simulink model "QuadcopterSimModel_Loiter_FTC_dseg"  (R2026a)
settings: Solver=ode2  StartTime=-5  StopTime=25  FixedStep=1/800  RelTol=1e-4  EnableMultiTasking=on
undefined symbols (not defined in the file): alt_ground, atmosphere, dseg_stop_en, envir, failure_time_mot_1, failure_time_mot_2, failure_time_mot_3, failure_time_mot_4, ffpar, g, pos_ref, westpar, wind
libraries: unit_conversions_lib x3, flightgear_visualization_lib x2, copterFtc_lib x2, atmosphere_lib x1, sensors_lib x1, quadcopter_lib x1, axes_transformation_lib x1
settings Model: Creator=Yannic  LastModifiedBy=wngh2
settings SolverCC: ZeroCrossControl=DisableAll
settings OptimizationCC: EfficientMapNaN2IntZero=off
settings DebuggingCC: ReadBeforeWriteMsg=DisableAll  WriteAfterWriteMsg=DisableAll  WriteAfterReadMsg=DisableAll  MultiTaskDSMMsg=none  MultiTaskRateTransMsg=warning
settings HardwareCC: TargetBitPerPointer=64.0  TargetBitPerSizeT=64.0  TargetBitPerPtrDiffT=64.0  TargetLongLongMode=on  TargetIntDivRoundTo=Zero  TargetEndianess=LittleEndian  TargetWordSize=64.0  TargetHWDeviceType=MATLAB Host  ProdEqTarget=off
settings SFSimCC: SFSimEcho=off
settings CodeAppCC: MaxIdLength=128.0
settings GRTTargetCC: CombineOutputUpdateFcns=off  GRTInterface=on

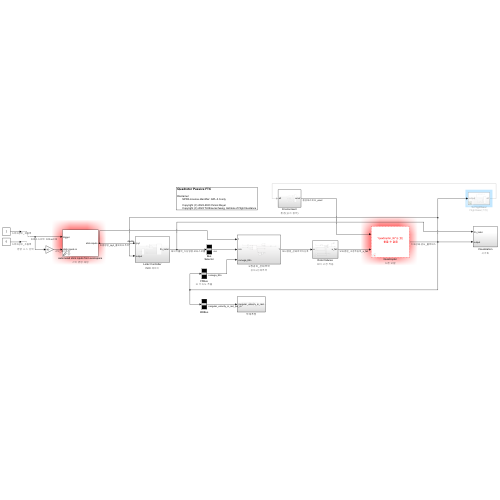
[thumbnail: Simulink's stored preview of the top-level diagram]
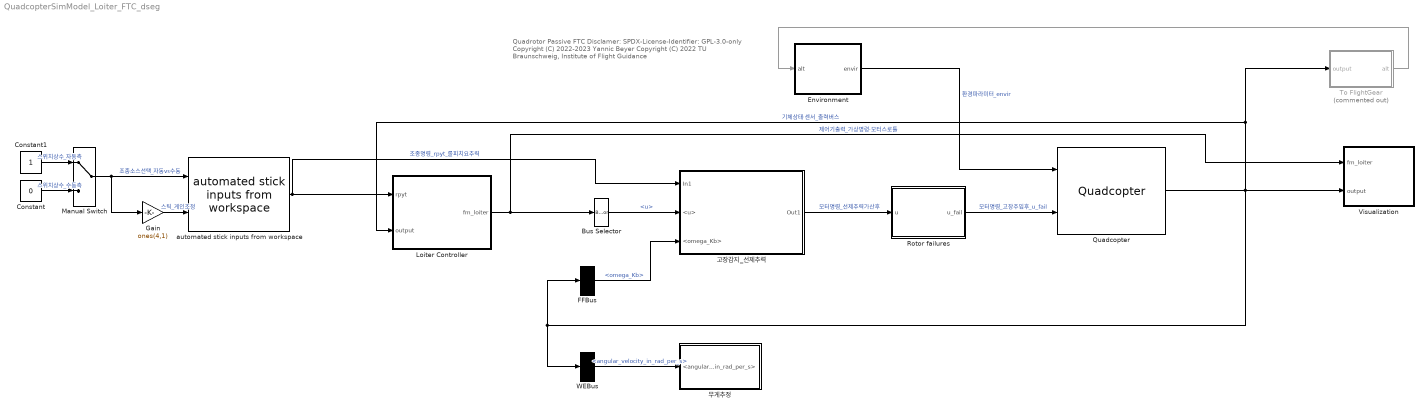
== system QuadcopterSimModel_Loiter_FTC_dseg ==
  note: Quadrotor Passive FTC
      |
      | Disclamer:
      | SPDX-License-Identifier: GPL-3.0-only
      |
      | Copyright (C) 2022-2023 Yannic Beyer
      | Copyright (C) 2022 TU Braunschweig, Institute of Flight Guidance
  Bus Selector : BusSelector  OutputSignals=inner_loop_indi.u
  Constant : Constant  Value=0
  Constant1 : Constant
  Environment : Subsystem  Description=고도 → 공기밀도·중력 등 환경 버스 계산
      settings: AttributesFormatString=환경(공기·중력)
  FFBus : BusSelector  Description=드론 상태 버스에서 요 각속도(omega_Kb) 추출 → 감지기로  OutputSignals=rigidBodyBus.omega_Kb
      settings: AttributesFormatString=요 각속도 추출
  Gain : Gain  Gain=ones(4,1)
  Loiter Controller : Subsystem  Description=INDI 로이터 제어기. 명령 + 피드백 → 모터 명령
      settings: AttributesFormatString=INDI 제어기
  Manual Switch : ManualSwitch  Description=명령 소스 선택 (sw=1: 자동 스틱 사용)
      settings: AttributesFormatString=명령 소스 선택
  Quadcopter : quadcopter_lib/Quadcopter  Description=드론 모델(동역학). 모터명령 → 힘·모멘트 → 상태(위치·자세·각속도)  copter_=copter  IC_=IC  grnd_=grnd
      settings: AttributesFormatString=드론 모델  SourceProductName=Quadcopter
  Rotor failures : Subsystem  Description=failure_time_mot_* 에 지정된 모터를 그 시각에 정지(스로틀 0)
      settings: AttributesFormatString=모터 고장 적용
  To FlightGear : Subsystem  Description=FlightGear 연동 (주석처리 — MATLAB Coder 필요)  Commented=on
      settings: AttributesFormatString=FlightGear(꺼짐)
  Visualization : Subsystem  Description=상태 시각화 출력
      settings: AttributesFormatString=시각화
  WEBus : BusSelector  OutputSignals=motorBus.angular_velocity_in_rad_per_s
  automated stick inputs from workspace : copterFtc_lib/automated stick inputs from workspace  Description=스틱 명령(simin) 재생 → rpyt 4채널(롤·피치·요·스로틀)  simin=simin
      settings: AttributesFormatString=스틱 명령 재생
  고장감지_선제추력 : Subsystem  Description=요 추종오차로 고장 감지 → 잔여 모터에 선제추력 주입 (감지·판단·주입 한 묶음)
      settings: AttributesFormatString=감지+선제추력
  무게추정 : Subsystem
  wires:
  Environment/1(envir) -> Quadcopter/1  "환경파라미터_envir"
  Quadcopter/1 -> To FlightGear/1(output), Loiter Controller/2(output), Visualization/2(output), FFBus/1, WEBus/1  "기체상태·센서_출력버스"
  To FlightGear/1(alt) -> Environment/1(alt)
  Rotor failures/1(u_fail) -> Quadcopter/2  "모터명령_고장주입후_u_fail"
  Loiter Controller/1(fm_loiter) -> Visualization/1(fm_loiter), Bus Selector/1  "제어기출력_가상명령·모터스로틀"
  automated stick inputs from workspace/1 -> 고장감지_선제추력/1(In1), Loiter Controller/1(rpyt)  "조종명령_rpyt_롤피치요추력"
  Constant1/1 -> Manual Switch/1  "스위치상수_자동측"
  Manual Switch/1 -> Gain/1, automated stick inputs from workspace/1  "조종소스선택_자동vs수동"
  Constant/1 -> Manual Switch/2  "스위치상수_수동측"
  Gain/1 -> automated stick inputs from workspace/2  "스틱_게인조정"
  Bus Selector/1 -> 고장감지_선제추력/2(<u>)  "<u>"
  FFBus/1 -> 고장감지_선제추력/3(<omega_Kb>)  "<omega_Kb>"
  고장감지_선제추력/1(Out1) -> Rotor failures/1(u)  "모터명령_선제추력가산후"
  WEBus/1 -> 무게추정/1(<angular_velocity_in_rad_per_s>)  "<angular_velocity_in_rad_per_s>"

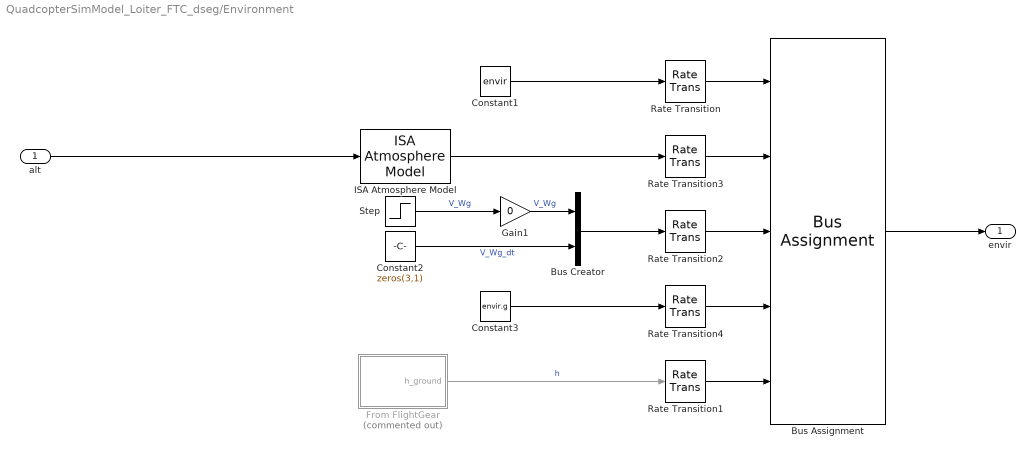
== system QuadcopterSimModel_Loiter_FTC_dseg/Environment ==
  alt : Inport
  Bus Assignment : BusAssignment  AssignedSignals=atmosphere,wind,g,alt_ground
  Bus Creator : BusCreator  Inputs=2
  Constant1 : Constant  Value=envir  OutDataTypeStr=Bus: envirBus
  Constant2 : Constant  Value=zeros(3,1)
  Constant3 : Constant  Value=envir.g
  From FlightGear : Subsystem  Commented=on
  Gain1 : Gain  Gain=0
  ISA Atmosphere Model : atmosphere_lib/ISA Atmosphere Model
      settings: SourceProductName=Atmosphere
  Rate Transition{,1..4} (5 alike) : RateTransition
  Step : Step  Time=3  FinalValue=[0;10;0]  SampleTime=0
  envir : Outport  VectorParamsAs1DForOutWhenUnconnected=off
  wires:
  From FlightGear/1(h_ground) -> Rate Transition1/1  "h"
  Rate Transition2/1 -> Bus Assignment/3
  Rate Transition3/1 -> Bus Assignment/2
  Bus Assignment/1 -> envir/1
  Rate Transition/1 -> Bus Assignment/1
  ISA Atmosphere Model/1 -> Rate Transition3/1
  Rate Transition1/1 -> Bus Assignment/5
  Constant1/1 -> Rate Transition/1
  alt/1 -> ISA Atmosphere Model/1
  Bus Creator/1 -> Rate Transition2/1
  Constant2/1 -> Bus Creator/2  "V_Wg_dt"
  Rate Transition4/1 -> Bus Assignment/4
  Constant3/1 -> Rate Transition4/1
  Gain1/1 -> Bus Creator/1  "V_Wg"
  Step/1 -> Gain1/1  "V_Wg"

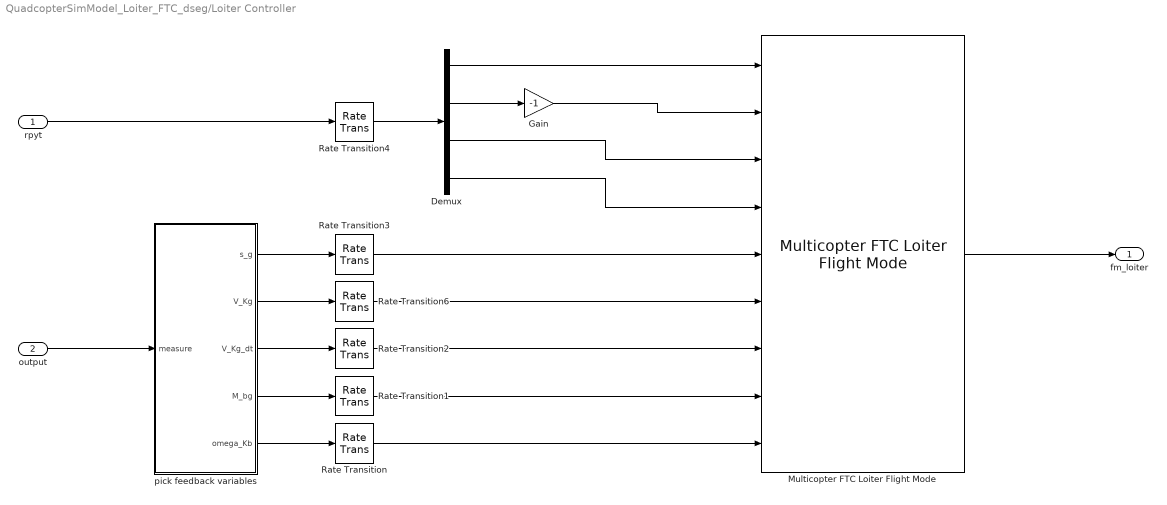
== system QuadcopterSimModel_Loiter_FTC_dseg/Loiter Controller ==
  rpyt : Inport  OutDataTypeStr=double
  output : Inport  Port=2
  Demux : Demux
  Gain : Gain  Gain=-1
  Multicopter FTC Loiter Flight Mode : copterFtc_lib/Multicopter FTC Loiter Flight Mode  fm=fm_loiter
  Rate Transition{,1..4,6} (6 alike) : RateTransition
  pick feedback variables : Subsystem
  fm_loiter : Outport  VectorParamsAs1DForOutWhenUnconnected=off
  wires:
  output/1 -> pick feedback variables/1(measure)
  rpyt/1 -> Rate Transition4/1
  Multicopter FTC Loiter Flight Mode/1 -> fm_loiter/1
  Demux/4 -> Multicopter FTC Loiter Flight Mode/4
  Demux/3 -> Multicopter FTC Loiter Flight Mode/3
  Demux/2 -> Gain/1
  Demux/1 -> Multicopter FTC Loiter Flight Mode/1
  Gain/1 -> Multicopter FTC Loiter Flight Mode/2
  Rate Transition4/1 -> Demux/1
  pick feedback variables/1(s_g) -> Rate Transition3/1
  pick feedback variables/5(omega_Kb) -> Rate Transition/1
  pick feedback variables/4(M_bg) -> Rate Transition1/1
  pick feedback variables/3(V_Kg_dt) -> Rate Transition2/1
  pick feedback variables/2(V_Kg) -> Rate Transition6/1
  Rate Transition/1 -> Multicopter FTC Loiter Flight Mode/9
  Rate Transition3/1 -> Multicopter FTC Loiter Flight Mode/5
  Rate Transition6/1 -> Multicopter FTC Loiter Flight Mode/6
  Rate Transition2/1 -> Multicopter FTC Loiter Flight Mode/7
  Rate Transition1/1 -> Multicopter FTC Loiter Flight Mode/8

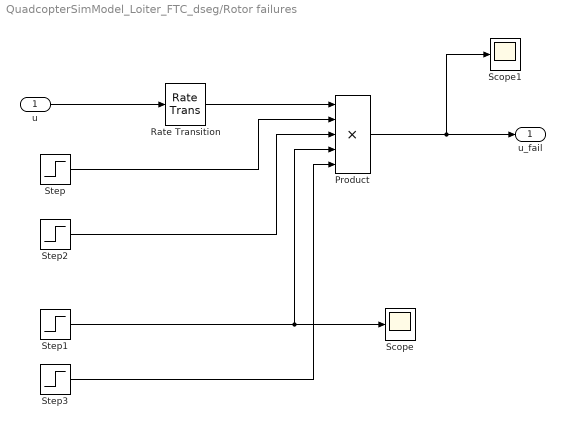
== system QuadcopterSimModel_Loiter_FTC_dseg/Rotor failures ==
  u : Inport
  Product : Product  Inputs=5
  Rate Transition : RateTransition
  Scope : Scope
      settings: ActiveDisplayYMinimum=-0.125  ActiveDisplayYMaximum=1.125  DataLoggingVariableName=ScopeData2
  Scope1 : Scope
      settings: ActiveDisplayYMinimum=-0.07201  ActiveDisplayYMaximum=0.64813
  Step : Step  Time=failure_time_mot_1  InitialValue=[1;1;1;1]  FinalValue=[0;1;1;1]  SampleTime=0
  Step1 : Step  Time=failure_time_mot_3  InitialValue=[1;1;1;1]  FinalValue=[1;1;0;1]  SampleTime=0
  Step2 : Step  Time=failure_time_mot_2  InitialValue=[1;1;1;1]  FinalValue=[1;0;1;1]  SampleTime=0
  Step3 : Step  Time=failure_time_mot_4  InitialValue=[1;1;1;1]  FinalValue=[1;1;1;0]  SampleTime=0
  u_fail : Outport  VectorParamsAs1DForOutWhenUnconnected=off
  wires:
  Product/1 -> Scope1/1, u_fail/1
  u/1 -> Rate Transition/1
  Rate Transition/1 -> Product/1
  Step1/1 -> Scope/1, Product/4
  Step2/1 -> Product/3
  Step/1 -> Product/2
  Step3/1 -> Product/5

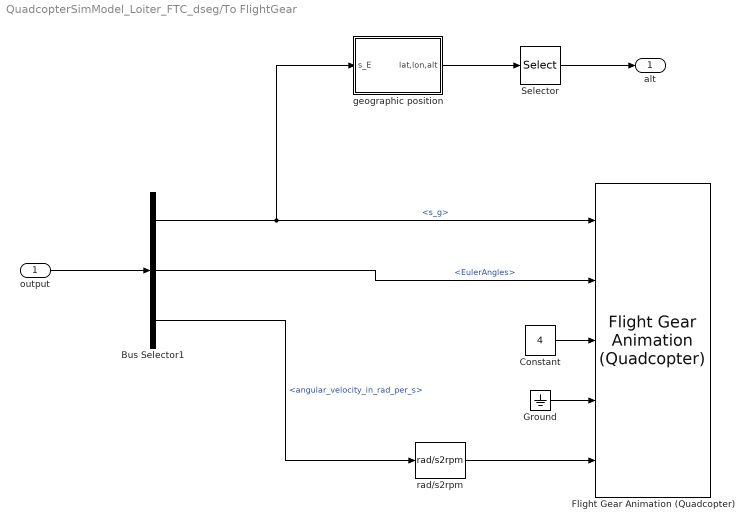
== system QuadcopterSimModel_Loiter_FTC_dseg/To FlightGear ==
  output : Inport
  Bus Selector1 : BusSelector  OutputSignals=rigidBodyBus.s_g,rigidBodyBus.EulerAngles,motorBus.angular_velocity_in_rad_per_s
  Constant : Constant  Value=4
  Flight Gear Animation (Quadcopter) : flightgear_visualization_lib/Flight Gear Animation (Quadcopter)  inital_lat=pos_ref.lat  inital_long=pos_ref.lon  inital_height=pos_ref.alt  remoteURL=fg.remoteURL  remotePort=fg.remotePort
      settings: SourceProductName=LADAC
  Ground : Ground
  Selector : Selector  InputPortWidth=3  IndexOptions=Index vector (dialog)  Indices=3  OutputSizes=1
  geographic position : Subsystem
  rad/s2rpm : unit_conversions_lib/rad//s2rpm
      settings: SourceProductName=LADAC
  alt : Outport  VectorParamsAs1DForOutWhenUnconnected=off
  wires:
  Bus Selector1/1 -> geographic position/1(s_E), Flight Gear Animation (Quadcopter)/1  "<s_g>"
  output/1 -> Bus Selector1/1
  geographic position/1(lat,lon,alt) -> Selector/1
  Bus Selector1/2 -> Flight Gear Animation (Quadcopter)/2  "<EulerAngles>"
  Bus Selector1/3 -> rad/s2rpm/1  "<angular_velocity_in_rad_per_s>"
  Selector/1 -> alt/1
  Constant/1 -> Flight Gear Animation (Quadcopter)/3
  Ground/1 -> Flight Gear Animation (Quadcopter)/4
  rad/s2rpm/1 -> Flight Gear Animation (Quadcopter)/5

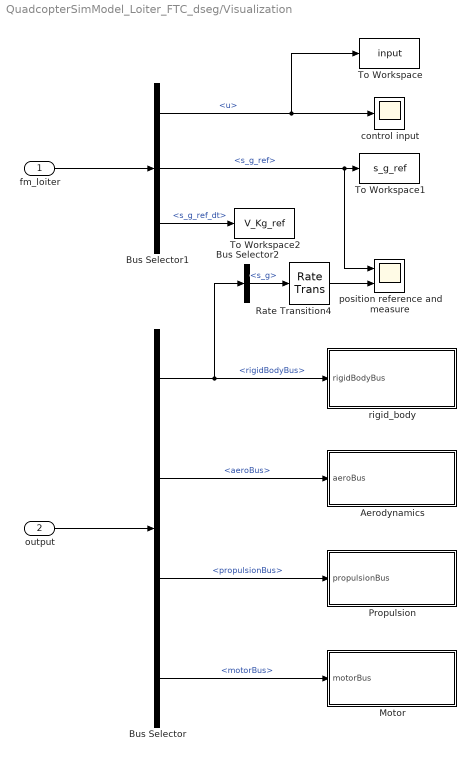
== system QuadcopterSimModel_Loiter_FTC_dseg/Visualization ==
  fm_loiter : Inport
  output : Inport  Port=2
  Aerodynamics : Subsystem
  Bus Selector : BusSelector  OutputSignals=rigidBodyBus,aeroBus,propulsionBus,motorBus
  Bus Selector1 : BusSelector  OutputSignals=inner_loop_indi.u,pos_cntrl.reference.s_g_ref,pos_cntrl.reference.s_g_ref_dt
  Bus Selector2 : BusSelector  OutputSignals=s_g
  Motor : Subsystem
  Propulsion : Subsystem
  Rate Transition4 : RateTransition
  To Workspace : ToWorkspace  VariableName=input  SaveFormat=Timeseries  SampleTime=-1
  To Workspace1 : ToWorkspace  VariableName=s_g_ref  SaveFormat=Timeseries  SampleTime=-1
  To Workspace2 : ToWorkspace  VariableName=V_Kg_ref  SaveFormat=Timeseries  SampleTime=-1
  control input : Scope
      settings: ActiveDisplayYMinimum=-0.0125  ActiveDisplayYMaximum=1.1125  DataLoggingVariableName=input
  position reference and measure : Scope  NumInputPorts=2
      settings: ActiveDisplayYMinimum=-0.60348  ActiveDisplayYMaximum=3.15627  DataLoggingVariableName=pos
  rigid_body : Subsystem
  wires:
  output/1 -> Bus Selector/1
  Bus Selector/1 -> Bus Selector2/1, rigid_body/1(rigidBodyBus)  "<rigidBodyBus>"
  Bus Selector/2 -> Aerodynamics/1(aeroBus)  "<aeroBus>"
  Bus Selector/3 -> Propulsion/1(propulsionBus)  "<propulsionBus>"
  Bus Selector/4 -> Motor/1(motorBus)  "<motorBus>"
  fm_loiter/1 -> Bus Selector1/1
  Bus Selector1/1 -> control input/1, To Workspace/1  "<u>"
  Bus Selector2/1 -> Rate Transition4/1  "<s_g>"
  Bus Selector1/2 -> position reference and measure/1, To Workspace1/1  "<s_g_ref>"
  Rate Transition4/1 -> position reference and measure/2
  Bus Selector1/3 -> To Workspace2/1  "<s_g_ref_dt>"

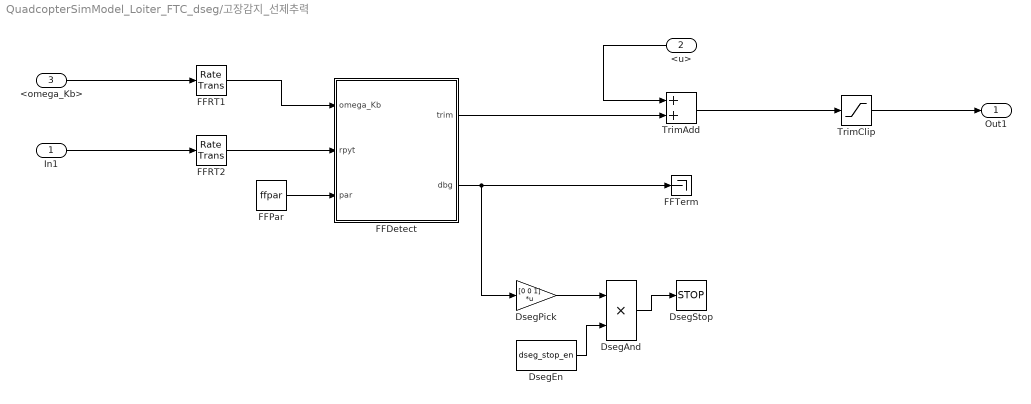
== system QuadcopterSimModel_Loiter_FTC_dseg/고장감지_선제추력 ==
  In1 : Inport
  <u> : Inport  Port=2
  <omega_Kb> : Inport  Port=3
  DsegAnd : Product
  DsegEn : Constant  Value=dseg_stop_en
  DsegPick : Gain  Gain=[0 0 1]  Multiplication=Matrix(K*u)
  DsegStop : Stop
  FFDetect : MATLAB Function  Description=감지·판단·주입 상태기계. |요오차|≥임계가 nper회 연속 → 고장 확정 → 주입 모터에 delta 선제추력  TreatAsAtomicUnit=on
      settings: AttributesFormatString=감지·판단·주입
  FFPar : Constant  Description=감지·주입 파라미터 ffpar (임계·주입량·주입 모터 마스크 등)  Value=ffpar  SampleTime=0.0025
      settings: AttributesFormatString=파라미터
  FFRT1 : RateTransition  Description=요 각속도를 감지 주기(400Hz)로 레이트 변환(연속→이산)  OutPortSampleTime=0.0025
      settings: AttributesFormatString=요율 레이트변환
  FFRT2 : RateTransition  Description=스틱 명령을 감지 주기로 레이트 변환  OutPortSampleTime=0.0025
      settings: AttributesFormatString=스틱 레이트변환
  FFTerm : Terminator
      settings: Description=감지 상태 로그(dbg) 종단  AttributesFormatString=로그 종단
  TrimAdd : Sum  Description=원래 모터 명령 + 선제추력 trim (건강한 모터 스로틀 상승)
      settings: AttributesFormatString=명령+선제추력
  TrimClip : Saturate  Description=합친 명령을 0~1로 클립(스로틀 물리 한계)  UpperLimit=1  LowerLimit=0
      settings: AttributesFormatString=0~1 클립
  Out1 : Outport
  wires:
  FFPar/1 -> FFDetect/3(par)
  <omega_Kb>/1 -> FFRT1/1
  In1/1 -> FFRT2/1
  FFRT2/1 -> FFDetect/2(rpyt)
  FFRT1/1 -> FFDetect/1(omega_Kb)
  FFDetect/2(dbg) -> FFTerm/1, DsegPick/1
  FFDetect/1(trim) -> TrimAdd/2
  TrimAdd/1 -> TrimClip/1
  <u>/1 -> TrimAdd/1
  TrimClip/1 -> Out1/1
  DsegPick/1 -> DsegAnd/1
  DsegEn/1 -> DsegAnd/2
  DsegAnd/1 -> DsegStop/1

== system QuadcopterSimModel_Loiter_FTC_dseg/무게추정 ==
  <angular_velocity_in_rad_per_s> : Inport
  WEClk : DigitalClock  SampleTime=0.0025
  WEPar : Constant  Value=westpar  SampleTime=0.0025
  WERT : RateTransition  OutPortSampleTime=0.0025
  WETerm : Terminator
  WeightEst : MATLAB Function  TreatAsAtomicUnit=on
  wires:
  WeightEst/1(mest) -> WETerm/1
  WEPar/1 -> WeightEst/3(par)
  <angular_velocity_in_rad_per_s>/1 -> WERT/1
  WERT/1 -> WeightEst/1(omega)
  WEClk/1 -> WeightEst/2(t)

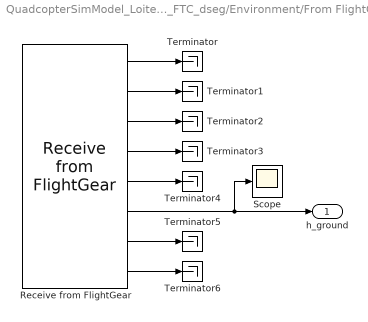
== system QuadcopterSimModel_Loiter_FTC_dseg/Environment/From FlightGear ==
  Receive from FlightGear : flightgear_visualization_lib/Receive from FlightGear  ip_address='127.0.0.1'  ip_port=5503  sample_time=1/8  blocking_time=0  is_aerocntrl=off  is_engine=off  is_fuel=off  is_land=off  is_avionics=off  is_envir=on
      settings: SourceProductName=LADAC
  Scope : Scope
      settings: ActiveDisplayYMinimum=4.70605  ActiveDisplayYMaximum=6.70605
  Terminator{,1..6} (7 alike) : Terminator
  h_ground : Outport  VectorParamsAs1DForOutWhenUnconnected=off
  wires:
  Receive from FlightGear/4 -> Terminator3/1
  Receive from FlightGear/5 -> Terminator4/1
  Receive from FlightGear/2 -> Terminator1/1
  Receive from FlightGear/7 -> Terminator5/1
  Receive from FlightGear/1 -> Terminator/1
  Receive from FlightGear/3 -> Terminator2/1
  Receive from FlightGear/8 -> Terminator6/1
  Receive from FlightGear/6 -> Scope/1, h_ground/1

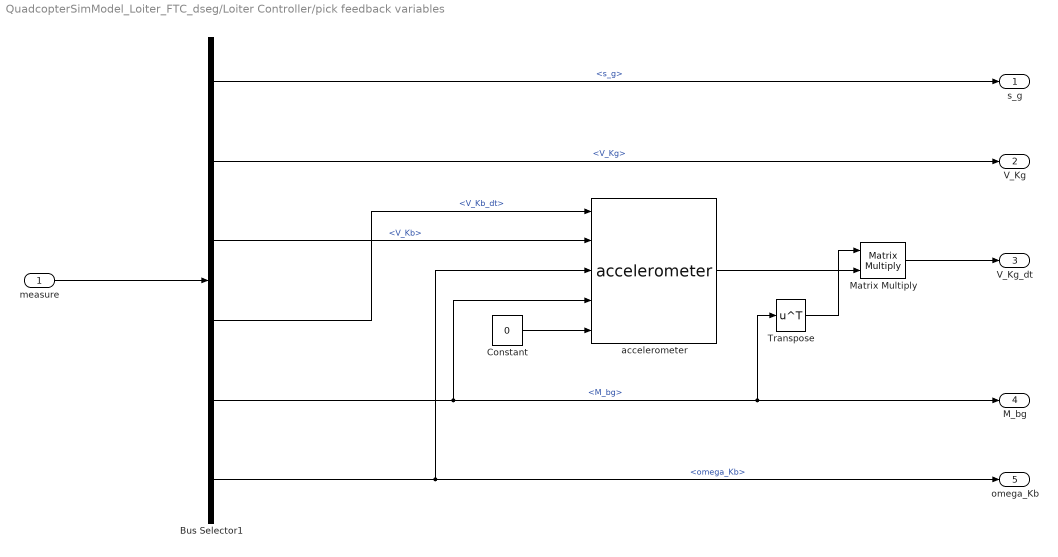
== system QuadcopterSimModel_Loiter_FTC_dseg/Loiter Controller/pick feedback variables ==
  measure : Inport
  Bus Selector1 : BusSelector  OutputSignals=rigidBodyBus.s_g,rigidBodyBus.V_Kg,rigidBodyBus.V_Kb,rigidBodyBus.V_Kb_dt,rigidBodyBus.M_bg,rigidBodyBus.omega_Kb
  Constant : Constant  Value=0
  Matrix Multiply : Product  Multiplication=Matrix(*)
  Transpose : Math  Operator=transpose  SignedPower=on
  accelerometer : sensors_lib/accelerometer  SystemSampleTime=-1  VariantActivationTime=update diagram  EmptyChoice=off  PassThrough=off  PassThroughVariantControl=(default)  EmptyChoiceVariantControl=(default)  AllowFlexibleInterface=on  Latency=0  AutoFrameSizeCalculation=off
      settings: SourceProductName=Sensors
  s_g : Outport  VectorParamsAs1DForOutWhenUnconnected=off
  V_Kg : Outport  Port=2  VectorParamsAs1DForOutWhenUnconnected=off
  V_Kg_dt : Outport  Port=3  VectorParamsAs1DForOutWhenUnconnected=off
  M_bg : Outport  Port=4  VectorParamsAs1DForOutWhenUnconnected=off
  omega_Kb : Outport  Port=5  VectorParamsAs1DForOutWhenUnconnected=off
  wires:
  measure/1 -> Bus Selector1/1
  Bus Selector1/4 -> accelerometer/1  "<V_Kb_dt>"
  accelerometer/1 -> Matrix Multiply/2
  Bus Selector1/1 -> s_g/1  "<s_g>"
  Bus Selector1/2 -> V_Kg/1  "<V_Kg>"
  Bus Selector1/5 -> Transpose/1, M_bg/1, accelerometer/4  "<M_bg>"
  Bus Selector1/6 -> omega_Kb/1, accelerometer/3  "<omega_Kb>"
  Constant/1 -> accelerometer/5
  Bus Selector1/3 -> accelerometer/2  "<V_Kb>"
  Matrix Multiply/1 -> V_Kg_dt/1
  Transpose/1 -> Matrix Multiply/1

== system QuadcopterSimModel_Loiter_FTC_dseg/To FlightGear/geographic position ==
  s_E : Inport
  Constant : Constant  Value=pos_ref.lat
  Constant1 : Constant  Value=pos_ref.lon
  Constant2 : Constant  Value=pos_ref.alt
  Mux : Mux  Inputs=3
  Scope : Scope  NumInputPorts=3
      settings: ActiveDisplayYMinimum=4.04731  ActiveDisplayYMaximum=63.57425  DataLoggingVariableName=ScopeData6
  "flat earth to lat, lon, alt" : axes_transformation_lib/NED to lat, lon, alt  SystemSampleTime=-1
      settings: SourceProductName=LADAC
  lat,lon,alt : Outport  VectorParamsAs1DForOutWhenUnconnected=off
  wires:
  Constant2/1 -> "flat earth to lat, lon, alt"/3
  Constant1/1 -> "flat earth to lat, lon, alt"/2
  "flat earth to lat, lon, alt"/3 -> Scope/3, Mux/3
  Constant/1 -> "flat earth to lat, lon, alt"/1
  Mux/1 -> lat,lon,alt/1
  s_E/1 -> "flat earth to lat, lon, alt"/4
  "flat earth to lat, lon, alt"/2 -> Mux/2, Scope/2
  "flat earth to lat, lon, alt"/1 -> Mux/1, Scope/1

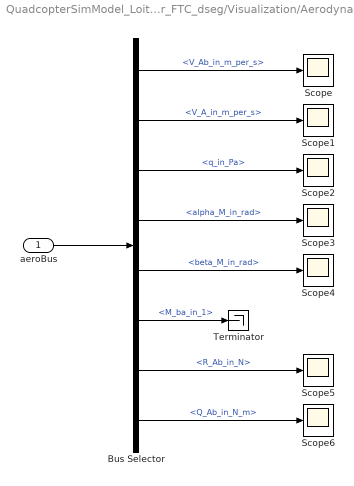
== system QuadcopterSimModel_Loiter_FTC_dseg/Visualization/Aerodynamics ==
  aeroBus : Inport
  Bus Selector : BusSelector  OutputSignals=V_Ab_in_m_per_s,V_A_in_m_per_s,q_in_Pa,angles.alpha_M_in_rad,angles.beta_M_in_rad,M_ba_in_1,R_Ab_in_N,Q_Ab_in_N_m
  Scope{,1..6} (7 alike) : Scope
      Scope1 settings: ActiveDisplayYMinimum=-0.81438  ActiveDisplayYMaximum=7.32941  DataLoggingVariableName=ScopeData2
      Scope2 settings: ActiveDisplayYMinimum=-7.65547  ActiveDisplayYMaximum=68.89921  DataLoggingVariableName=ScopeData3
      Scope3 settings: ActiveDisplayYMinimum=-0.08528  ActiveDisplayYMaximum=-0.00577  DataLoggingVariableName=ScopeData4
      Scope4 settings: ActiveDisplayYMinimum=-3.92698  ActiveDisplayYMaximum=3.92696  DataLoggingVariableName=ScopeData5
      Scope5 settings: ActiveDisplayYMinimum=-0.98924  ActiveDisplayYMaximum=1.67644  DataLoggingVariableName=ScopeData6
      Scope6 settings: ActiveDisplayYMinimum=-0.00019  ActiveDisplayYMaximum=2E-5  DataLoggingVariableName=ScopeData7
  Terminator : Terminator
  wires:
  aeroBus/1 -> Bus Selector/1
  Bus Selector/1 -> Scope/1  "<V_Ab_in_m_per_s>"
  Bus Selector/2 -> Scope1/1  "<V_A_in_m_per_s>"
  Bus Selector/3 -> Scope2/1  "<q_in_Pa>"
  Bus Selector/4 -> Scope3/1  "<alpha_M_in_rad>"
  Bus Selector/5 -> Scope4/1  "<beta_M_in_rad>"
  Bus Selector/6 -> Terminator/1  "<M_ba_in_1>"
  Bus Selector/7 -> Scope5/1  "<R_Ab_in_N>"
  Bus Selector/8 -> Scope6/1  "<Q_Ab_in_N_m>"

== system QuadcopterSimModel_Loiter_FTC_dseg/Visualization/Motor ==
  motorBus : Inport
  Bus Selector : BusSelector  OutputSignals=angular_acceleration_in_rad_per_square_s,angular_velocity_in_rad_per_s
  Scope : Scope
      settings: ActiveDisplayYMinimum=-14601.27633  ActiveDisplayYMaximum=1999.66838  DataLoggingVariableName=ScopeData15
  Scope1 : Scope
      settings: ActiveDisplayYMinimum=-467.75743  ActiveDisplayYMaximum=3230.1471  DataLoggingVariableName=motor_speed
  To Workspace : ToWorkspace  VariableName=motor_speed  SaveFormat=Timeseries  SampleTime=-1
  wires:
  Bus Selector/1 -> Scope/1  "<angular_acceleration_in_rad_per_square_s>"
  motorBus/1 -> Bus Selector/1
  Bus Selector/2 -> To Workspace/1, Scope1/1  "<angular_velocity_in_rad_per_s>"

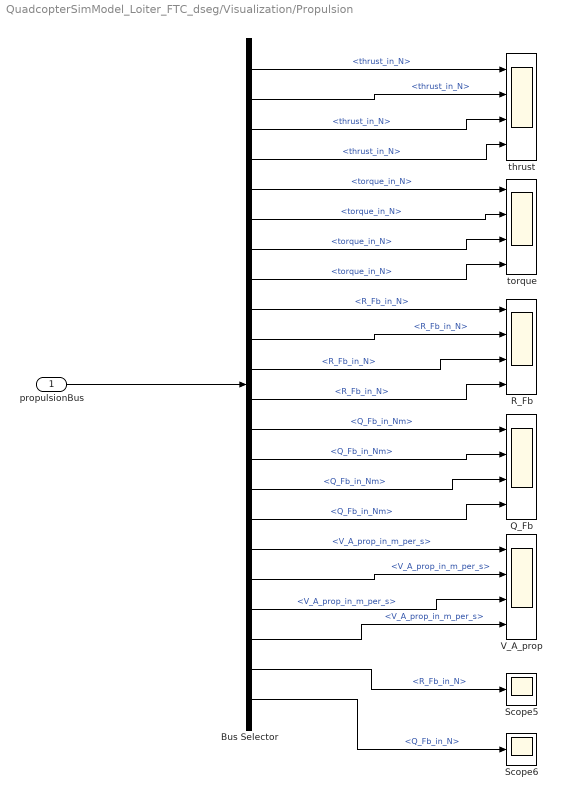
== system QuadcopterSimModel_Loiter_FTC_dseg/Visualization/Propulsion ==
  propulsionBus : Inport
  Bus Selector : BusSelector  OutputSignals=propeller_1.thrust_in_N,propeller_2.thrust_in_N,propeller_3.thrust_in_N,propeller_4.thrust_in_N,propeller_1.torque_in_N,propeller_2.torque_in_N,propeller_3.torque_in_N,propeller_4.torque_in_N,propeller_1.R_Fb_in_N,propeller_2.R_Fb_in_N,propeller_3.R_Fb_in_N,propeller_4.R_Fb_in_N,propeller_1.Q_Fb_in_Nm,propeller_2.Q_Fb_in_Nm,propeller_3.Q_Fb_in_Nm,propeller_4.Q_Fb_in_Nm,propeller_1.V_A_prop_in_m_per_s,propeller_2.V_A_prop_in_m_per_s,propeller_3.V_A_prop_in_m_per_s,propeller_4.V_A_prop_in_m_per_s,R_Fb_in_N,Q_Fb_in_N
  Q_Fb : Scope  NumInputPorts=4
      settings: ActiveDisplayYMinimum=-0.22601  ActiveDisplayYMaximum=-0.19277  DataLoggingVariableName=ScopeData11
  R_Fb : Scope  NumInputPorts=4
      settings: ActiveDisplayYMinimum=-8.5339  ActiveDisplayYMaximum=0.94821  DataLoggingVariableName=ScopeData10
  Scope5 : Scope
      settings: ActiveDisplayYMinimum=-20.94875  ActiveDisplayYMaximum=2.32764  DataLoggingVariableName=ScopeData13
  Scope6 : Scope
      settings: ActiveDisplayYMinimum=-0.90403  ActiveDisplayYMaximum=-0.77107  DataLoggingVariableName=ScopeData14
  V_A_prop : Scope  NumInputPorts=4
      settings: ActiveDisplayYMinimum=-0.02599  ActiveDisplayYMaximum=0.06439  DataLoggingVariableName=ScopeData12
  thrust : Scope  NumInputPorts=4
      settings: ActiveDisplayYMinimum=-0.01333  ActiveDisplayYMaximum=0.11998  DataLoggingVariableName=ScopeData8
  torque : Scope  NumInputPorts=4
      settings: ActiveDisplayYMinimum=-0.00039  ActiveDisplayYMaximum=0.00353  DataLoggingVariableName=ScopeData9
  wires:
  propulsionBus/1 -> Bus Selector/1
  Bus Selector/1 -> thrust/1  "<thrust_in_N>"
  Bus Selector/2 -> thrust/2  "<thrust_in_N>"
  Bus Selector/3 -> thrust/3  "<thrust_in_N>"
  Bus Selector/4 -> thrust/4  "<thrust_in_N>"
  Bus Selector/5 -> torque/1  "<torque_in_N>"
  Bus Selector/6 -> torque/2  "<torque_in_N>"
  Bus Selector/7 -> torque/3  "<torque_in_N>"
  Bus Selector/8 -> torque/4  "<torque_in_N>"
  Bus Selector/9 -> R_Fb/1  "<R_Fb_in_N>"
  Bus Selector/10 -> R_Fb/2  "<R_Fb_in_N>"
  Bus Selector/11 -> R_Fb/3  "<R_Fb_in_N>"
  Bus Selector/12 -> R_Fb/4  "<R_Fb_in_N>"
  Bus Selector/13 -> Q_Fb/1  "<Q_Fb_in_Nm>"
  Bus Selector/14 -> Q_Fb/2  "<Q_Fb_in_Nm>"
  Bus Selector/15 -> Q_Fb/3  "<Q_Fb_in_Nm>"
  Bus Selector/16 -> Q_Fb/4  "<Q_Fb_in_Nm>"
  Bus Selector/17 -> V_A_prop/1  "<V_A_prop_in_m_per_s>"
  Bus Selector/18 -> V_A_prop/2  "<V_A_prop_in_m_per_s>"
  Bus Selector/19 -> V_A_prop/3  "<V_A_prop_in_m_per_s>"
  Bus Selector/20 -> V_A_prop/4  "<V_A_prop_in_m_per_s>"
  Bus Selector/21 -> Scope5/1  "<R_Fb_in_N>"
  Bus Selector/22 -> Scope6/1  "<Q_Fb_in_N>"

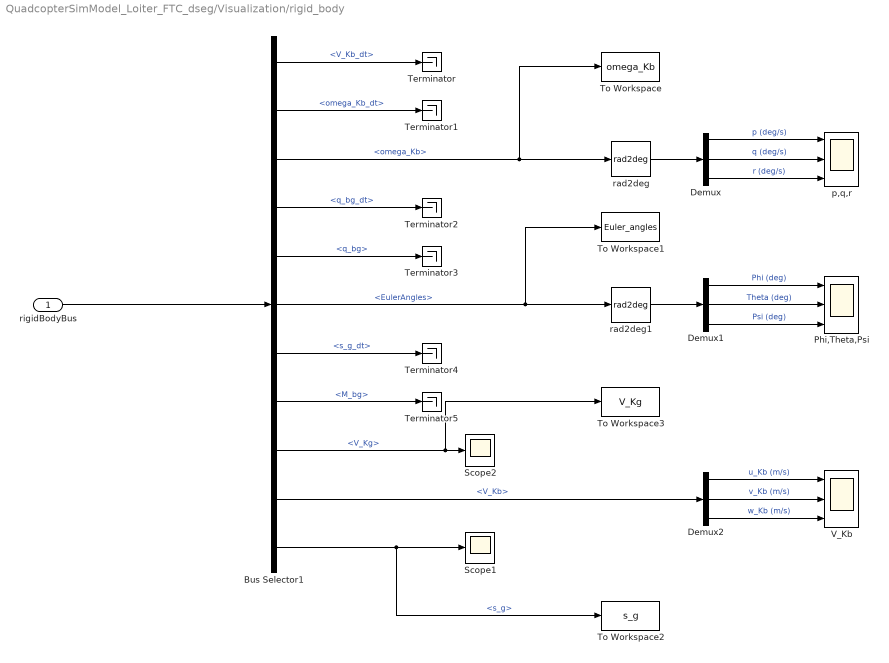
== system QuadcopterSimModel_Loiter_FTC_dseg/Visualization/rigid_body ==
  rigidBodyBus : Inport
  Bus Selector1 : BusSelector  OutputSignals=V_Kb_dt,omega_Kb_dt,omega_Kb,q_bg_dt,q_bg,EulerAngles,s_g_dt,M_bg,V_Kg,V_Kb,s_g
  Demux : Demux  Outputs=3
  Demux1 : Demux  Outputs=3
  Demux2 : Demux  Outputs=3
  Phi,Theta,Psi : Scope  NumInputPorts=3
      settings: ActiveDisplayYMinimum=-224.96763  ActiveDisplayYMaximum=224.97291  DataLoggingVariableName=ScopeAngles
  Scope1 : Scope
      settings: ActiveDisplayYMinimum=-1.80345  ActiveDisplayYMaximum=15.72277  DataLoggingVariableName=s_g
  Scope2 : Scope
      settings: ActiveDisplayYMinimum=-6.91604  ActiveDisplayYMaximum=6.91222
  Terminator{,1..5} (6 alike) : Terminator
  To Workspace : ToWorkspace  VariableName=omega_Kb  SaveFormat=Timeseries  SampleTime=-1
  To Workspace1 : ToWorkspace  VariableName=Euler_angles  SaveFormat=Timeseries  SampleTime=-1
  To Workspace2 : ToWorkspace  VariableName=s_g  SaveFormat=Timeseries  SampleTime=-1
  To Workspace3 : ToWorkspace  VariableName=V_Kg  SaveFormat=Timeseries  SampleTime=-1
  V_Kb : Scope  NumInputPorts=3
      settings: ActiveDisplayYMinimum=-13.81743  ActiveDisplayYMaximum=1.75322  DataLoggingVariableName=ScopeV
  p,q,r : Scope  NumInputPorts=3
      settings: ActiveDisplayYMinimum=-1779.61844  ActiveDisplayYMaximum=903.66048  DataLoggingVariableName=ScopeRates
  rad2deg : unit_conversions_lib/rad2deg
      settings: SourceProductName=Unit Conversions
  rad2deg1 : unit_conversions_lib/rad2deg
      settings: SourceProductName=Unit Conversions
  wires:
  Demux/1 -> p,q,r/1  "p (deg/s)"
  Demux1/2 -> Phi,Theta,Psi/2  "Theta (deg)"
  rad2deg/1 -> Demux/1
  Demux1/1 -> Phi,Theta,Psi/1  "Phi (deg)"
  Demux1/3 -> Phi,Theta,Psi/3  "Psi (deg)"
  Demux2/3 -> V_Kb/3  "w_Kb (m/s)"
  Bus Selector1/7 -> Terminator4/1  "<s_g_dt>"
  Bus Selector1/6 -> To Workspace1/1, rad2deg1/1  "<EulerAngles>"
  Bus Selector1/3 -> To Workspace/1, rad2deg/1  "<omega_Kb>"
  Demux/3 -> p,q,r/3  "r (deg/s)"
  Bus Selector1/1 -> Terminator/1  "<V_Kb_dt>"
  Demux2/2 -> V_Kb/2  "v_Kb (m/s)"
  Demux/2 -> p,q,r/2  "q (deg/s)"
  rad2deg1/1 -> Demux1/1
  Bus Selector1/5 -> Terminator3/1  "<q_bg>"
  Demux2/1 -> V_Kb/1  "u_Kb (m/s)"
  Bus Selector1/10 -> Demux2/1  "<V_Kb>"
  rigidBodyBus/1 -> Bus Selector1/1
  Bus Selector1/8 -> Terminator5/1  "<M_bg>"
  Bus Selector1/4 -> Terminator2/1  "<q_bg_dt>"
  Bus Selector1/2 -> Terminator1/1  "<omega_Kb_dt>"
  Bus Selector1/9 -> To Workspace3/1, Scope2/1  "<V_Kg>"
  Bus Selector1/11 -> To Workspace2/1, Scope1/1  "<s_g>"

== matlab function QuadcopterSimModel_Loiter_FTC_dseg/무게추정/WeightEst ==
  data: omega input; mest output; t input; par input
function mest = WeightEst(omega, t, par)
%#codegen
persistent acc n val done
if isempty(acc), acc = 0; n = 0; val = 0; done = false; end
m_dry = par(1);  ss_dry = par(2);  t0 = par(3);  t1 = par(4);
if ~done && t >= t0 && t <= t1
    acc = acc + sum(omega.^2);
    n   = n + 1;
end
if ~done && t > t1 && n > 0
    val  = m_dry*(acc/n)/ss_dry - m_dry;
    done = true;
end
mest = val;
end

== matlab function QuadcopterSimModel_Loiter_FTC_dseg/고장감지_선제추력/FFDetect ==
  data: omega_Kb input; trim output; rpyt input; par input; dbg output
function [trim, dbg] = FFDetect(omega_Kb, rpyt, par)
%#codegen
persistent rref cnt state cff mk
if isempty(rref), rref = 0; cnt = 0; state = 0; cff = 0; mk = zeros(4,1); end
delta = par(1);  th = par(2);  nper = par(3);  nff = par(4);
rmax  = par(5);  rtc = par(6); ts   = par(7);  mask = par(8:11);
r   = omega_Kb(3) * 180/pi;
tgt = rpyt(3) * rmax;
a   = ts / (rtc + ts);
rref = rref + a*(tgt - rref);
e = r - rref;
if state == 0
    if abs(e) >= th, cnt = cnt + 1; else, cnt = 0; end
    if cnt >= nper
        state = 1; cff = 0;
        if any(mask ~= 0)
            mk = mask(:);
        elseif e > 0
            mk = [0; 1; 0; 1];
        else
            mk = [1; 0; 1; 0];
        end
    end
end
trim = zeros(4,1);
if state == 1
    trim = delta * mk;
    cff  = cff + 1;
    if cff >= nff, state = 2; end
end
dbg = [e; rref; double(state)];
end
